simulink model "sm_wheel_loader_driveline"  (R2025a)
settings: Solver=VariableStepAuto  StartTime=0.0  StopTime=20  RelTol=1e-3  AbsTol=1e-3  EnableMultiTasking=on
undefined symbols (not defined in the file or in its folder): Wheel_Loader, X, Y, Z
libraries: sm_lib x12, sm_wheel_loader_lib x6, nesl_utility x3, fl_lib x3
Description:
  | Copyright 2023-2025 The MathWorks, Inc.
settings Model: Creator=smiller  LastModifiedBy=smiller
settings SolverCC: AutoScaleAbsTol=off  AlgebraicLoopSolver=TrustRegion  MaxZcPerStep=1.0
settings DataIOCC: LimitDataPoints=on  MaxDataPoints=10000  ReturnWorkspaceOutputs=off  SignalLoggingName=logsout_sm_wheel_loader_driveline
settings OptimizationCC: ReuseModelBlockBuffer=off  LifeSpan=inf
settings DebuggingCC: UnconnectedInputMsg=warning  UnconnectedOutputMsg=warning  UnconnectedLineMsg=warning  AllowSymbolicDim=off  SubsystemReferenceDiagnosticForUnitTest=warning  SFUnexpectedBacktrackingDiag=warning  SFNoUnconditionalDefaultTransitionDiag=warning  SFExecutionAtInitializationDiag=none  ArithmeticOperatorsInVariantConditions=warning
settings ModelReferenceCC: EnableRefExpFcnMdlSchedulingChecks=on
settings SFSimCC: SimUseLocalCustomCode=off  CustomCodeUndefinedFunction=UseInterfaceOnly
settings RTWCC: RTWUseLocalCustomCode=off  GPUComputeCapability=3.5  DLArmComputeVersion=19.05
settings CodeAppCC: StateflowObjectComments=on
settings GRTTargetCC: TargetLangStandard=C89/C90 (ANSI)
settings ConfigComp: CovMetricSettings=dw  CovSaveCumulativeToWorkspaceVar=on  CovSaveSingleToWorkspaceVar=on  CovExternalEMLEnable=off  CovSFcnEnable=off
settings SimscapeCC: SimscapeLogType=all  SimscapeLogSimulationStatistics=on  SimscapeLogName=simlog_sm_wheel_loader_driveline  SimscapeLogDataHistory=10000.0
settings DiagnosticsConfigSet: SimMechanicsUnconnectedFramePorts=none
settings ExplorerConfigSet: InternalSimMechanicsExplorerSettings="<ExplorerConfiguration><canonicalview>default</canonicalview><AnimationSetting><BasePlaybackSpeed>1.0</BasePlaybackSpeed><PlaybackSpeedFactor>1.0</PlaybackSpeedFactor></AnimationSetting><TilePanel><TileInfo><Tiles Columns=\"1\" Count=\"1\" Rows=\"1\"><Column Weight=\"1\"/><Row Weight=\"1\"/><Tile Height=\"1\" Width=\"1\" X=\"0\" Y=\"0\"/></Tiles></TileInfo><SceneInfo><SceneViewer><BGColor><R>1</R><G>1</G><B>1</B></BGColor><Camera><DoPerspective>off</DoPerspective><Position><X>-0.927464937859153515</X><Y>-0.882013825634648696</Y><Z>0.258089805407605677</Z></Position><Center><X>-0.254615293064785364</X><Y>-0.20835009329744858</Y><Z>-0.047606990836146286</Z></Center><Up><X>0.634087832148672037</X><Y>-0.738030275124983537</Y><Z>-0.230746471522185359</Z></Up><ViewLimDist>1</ViewLimDist><YLim>0.133380146481821338</YLim><XLim>0.282253946342844175</XLim></Camera></SceneViewer></SceneInfo></TilePanel><MechEditorPanel><Cameras/><GfxPanelCameraMap/><VideoCreator><PlaybackSpeedRatio>1.0</PlaybackSpeedRatio><FrameRate>30</FrameRate><VideoFormat>Motion JPEG AVI</VideoFormat><FrameSize>auto</FrameSize></VideoCreator></MechEditorPanel></ExplorerConfiguration>"

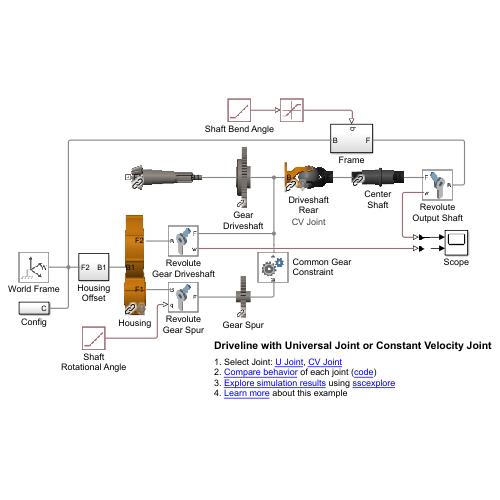
[thumbnail: Simulink's stored preview of the top-level diagram]
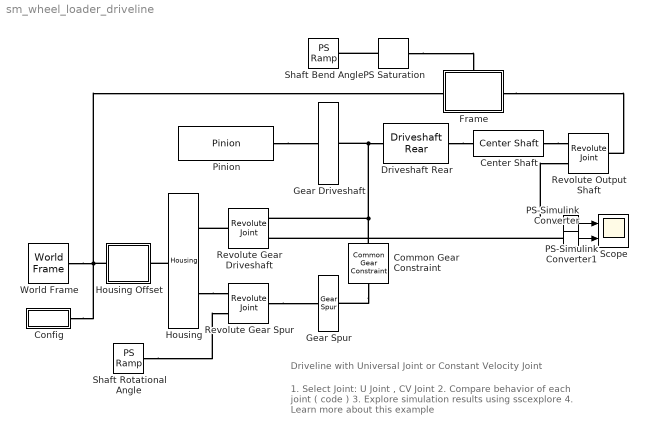
== system sm_wheel_loader_driveline ==
  note: Driveline with Universal Joint or Constant Velocity Joint
  note: 1. Select Joint: U Joint , CV Joint
      | 2. Compare behavior of each joint ( code )
      | 3. Explore simulation results using sscexplore
      | 4. Learn more about this example
  Center Shaft : sm_wheel_loader_lib/Wheel Loader Vehicle/Driveline/Driveline/Driveline 3D/Center Shaft  SystemSampleTime=-1  VariantActivationTime=update diagram  EmptyChoice=off  PassThrough=off  PassThroughVariantControl=(default)  EmptyChoiceVariantControl=(default)  AllowFlexibleInterface=on  Latency=0  AutoFrameSizeCalculation=off
  Common Gear Constraint : sm_lib/Gears and Couplings/Gears/Common Gear Constraint  GearType=External  SpecificationType=CenterDistanceRatio  CenterDistance=0.159173333333337  CenterDistanceUnits=m  GearRatio=60/34  BaseGearRadius=10.0  BaseGearRadiusUnits=cm  FollGearRadius=10.0  FollGearRadiusUnits=cm
  Config : Subsystem
  Driveshaft Rear : sm_wheel_loader_lib/Wheel Loader Vehicle/Driveline/Driveline/Driveline 3D/Driveshaft Rear  popup_driveJointR=CV Joint
      settings: AttributesFormatString=%<popup_driveJointR>
  Frame : Subsystem
      settings: PortSchema="{\"entries\":[{\"content\":{\"sides\":[{\"content\":{\"connectorIds\":[\"LConn1\"]},\"type\":\"ConnectorPlacement.EquallySpacedRectSide\",\"uuid\":\"e6cbbeaa-eea4-475d-99a8-9813de6a09fd\"},{\"content\":{\"connectorIds\":[\"RConn1\"],\"side\":\"RIGHT\"},\"type\":\"ConnectorPlacement.EquallySpacedRectSide\",\"uuid\":\"b42ffd92-551a-432a-a88e-4fe80a794cd4\"},{\"content\":{\"connectorIds\":[\"LConn2\"],\"side\":\"TOP\"},\"type\":\"ConnectorPlacement.EquallySpacedRectSide\",\"uuid\":\"5e4255e5-ca05-41fd-94c5-358a7ae7d752\"}]},\"type\":\"ConnectorPlacement.EquallySpacedConnector\",\"uuid\":\"ee1dc33c-92b2-4d9a-b7e0-7adfd33d81e9\"}],\"packageUris\":[\"http://schema.mathworks.com/mf0/Connector/R2020b\"],\"version\":\"1.0\"}"
  Gear Driveshaft : sm_wheel_loader_lib/Wheel Loader Vehicle/Driveline/Driveline/Driveline 3D/Gear Driveshaft  Tag=431AF5D6-54DA-7142-9431-C4596B630D74  SystemSampleTime=-1  VariantActivationTime=update diagram  EmptyChoice=off  PassThrough=off  PassThroughVariantControl=(default)  EmptyChoiceVariantControl=(default)  AllowFlexibleInterface=on  Latency=0  AutoFrameSizeCalculation=off
  Gear Spur : sm_wheel_loader_lib/Wheel Loader Vehicle/Driveline/Driveline/Driveline 3D/Gear Spur  Tag=6EB64544-2A1C-0847-BADC-74C9179BE488  SystemSampleTime=-1  VariantActivationTime=update diagram  EmptyChoice=off  PassThrough=off  PassThroughVariantControl=(default)  EmptyChoiceVariantControl=(default)  AllowFlexibleInterface=on  Latency=0  AutoFrameSizeCalculation=off
  Housing : sm_wheel_loader_lib/Wheel Loader Vehicle/Driveline/Driveline/Driveline 3D/Housing  Tag=FD1DF3FF-DA5A-0743-8F9C-61712535B657  finalDr_casing_opc=0.1
  Housing Offset : Subsystem
  PS Saturation : fl_lib/Physical Signals/Nonlinear Operators/PS Saturation  upper_limit=pi/4 rad  lower_limit=-pi/4 rad  ZeroCross=true
  PS-Simulink Converter : nesl_utility/PS-Simulink Converter  PhysicalDomain=network_engine_domain  SubClassName=ps_output  LeftPortType=input  RightPortType=output  PseudoPeriodic=off  Frequencies=[]  VectorFormat=inherit  Unit=inherit  AffineConversion=off
  PS-Simulink Converter1 : nesl_utility/PS-Simulink Converter  PhysicalDomain=network_engine_domain  SubClassName=ps_output  LeftPortType=input  RightPortType=output  PseudoPeriodic=off  Frequencies=[]  VectorFormat=inherit  Unit=inherit  AffineConversion=off
  Pinion : sm_wheel_loader_lib/Wheel Loader Vehicle/Driveline/Driveline/Driveline 3D/Pinion  Tag=8E104B94-12D7-814C-ADF4-87AC864C83F8  SystemSampleTime=-1  VariantActivationTime=update diagram  EmptyChoice=off  PassThrough=off  PassThroughVariantControl=(default)  EmptyChoiceVariantControl=(default)  AllowFlexibleInterface=on  Latency=0  AutoFrameSizeCalculation=off
  Revolute Gear Driveshaft : sm_lib/Joints/Revolute Joint  JointMode=Normal  CompositeWrenchDir=FollowerOnBase  CompositeWrenchFrame=BaseFrame  SenseConstraintForce=off  SenseConstraintTorque=off  SenseTotalForce=off  SenseTotalTorque=off  PositionTargetSpecify=off  PositionTargetPriority=High  PositionTargetValue=0  PositionTargetValueUnits=deg  VelocityTargetSpecify=off  VelocityTargetPriority=High  VelocityTargetValue=0  VelocityTargetValueUnits=deg/s  EquilibriumPosition=0  EquilibriumPositionUnits=deg  SpringStiffness=0  SpringStiffnessUnits=N*m/deg  DampingCoefficient=0  DampingCoefficientUnits=N*m/(deg/s)  LowerLimitSpecify=off  LowerLimitBound=-90  LowerLimitBoundUnits=deg  LowerLimitStiffness=1e4  LowerLimitStiffnessUnits=N*m/deg  LowerLimitDamping=10  LowerLimitDampingUnits=N*m/(deg/s)  LowerLimitTransitionRegionWidth=0.1  LowerLimitTransitionRegionWidthUnits=deg  UpperLimitSpecify=off  UpperLimitBound=90  UpperLimitBoundUnits=deg  UpperLimitStiffness=1e4  UpperLimitStiffnessUnits=N*m/deg  UpperLimitDamping=10  UpperLimitDampingUnits=N*m/(deg/s)  UpperLimitTransitionRegionWidth=0.1  UpperLimitTransitionRegionWidthUnits=deg  TorqueActuationMode=NoTorque  MotionActuationMode=ComputedMotion  SensePosition=off  SenseVelocity=on  SenseAcceleration=off  SenseTorqueForce=off  SenseLowerLimitTorqueForce=off  SenseUpperLimitTorqueForce=off
  Revolute Gear Spur : sm_lib/Joints/Revolute Joint  JointMode=Normal  CompositeWrenchDir=FollowerOnBase  CompositeWrenchFrame=BaseFrame  SenseConstraintForce=off  SenseConstraintTorque=off  SenseTotalForce=off  SenseTotalTorque=off  PositionTargetSpecify=off  PositionTargetPriority=High  PositionTargetValue=0  PositionTargetValueUnits=deg  VelocityTargetSpecify=off  VelocityTargetPriority=High  VelocityTargetValue=0  VelocityTargetValueUnits=deg/s  EquilibriumPosition=0  EquilibriumPositionUnits=deg  SpringStiffness=0  SpringStiffnessUnits=N*m/deg  DampingCoefficient=0  DampingCoefficientUnits=N*m/(deg/s)  LowerLimitSpecify=off  LowerLimitBound=-90  LowerLimitBoundUnits=deg  LowerLimitStiffness=1e4  LowerLimitStiffnessUnits=N*m/deg  LowerLimitDamping=10  LowerLimitDampingUnits=N*m/(deg/s)  LowerLimitTransitionRegionWidth=0.1  LowerLimitTransitionRegionWidthUnits=deg  UpperLimitSpecify=off  UpperLimitBound=90  UpperLimitBoundUnits=deg  UpperLimitStiffness=1e4  UpperLimitStiffnessUnits=N*m/deg  UpperLimitDamping=10  UpperLimitDampingUnits=N*m/(deg/s)  UpperLimitTransitionRegionWidth=0.1  UpperLimitTransitionRegionWidthUnits=deg  TorqueActuationMode=ComputedTorque  MotionActuationMode=InputMotion  SensePosition=off  SenseVelocity=off  SenseAcceleration=off  SenseTorqueForce=off  SenseLowerLimitTorqueForce=off  SenseUpperLimitTorqueForce=off
  Revolute Output Shaft : sm_lib/Joints/Revolute Joint  JointMode=Normal  CompositeWrenchDir=FollowerOnBase  CompositeWrenchFrame=BaseFrame  SenseConstraintForce=off  SenseConstraintTorque=off  SenseTotalForce=off  SenseTotalTorque=off  PositionTargetSpecify=off  PositionTargetPriority=High  PositionTargetValue=0  PositionTargetValueUnits=deg  VelocityTargetSpecify=off  VelocityTargetPriority=High  VelocityTargetValue=0  VelocityTargetValueUnits=deg/s  EquilibriumPosition=0  EquilibriumPositionUnits=deg  SpringStiffness=0  SpringStiffnessUnits=N*m/deg  DampingCoefficient=0  DampingCoefficientUnits=N*m/(deg/s)  LowerLimitSpecify=off  LowerLimitBound=-90  LowerLimitBoundUnits=deg  LowerLimitStiffness=1e4  LowerLimitStiffnessUnits=N*m/deg  LowerLimitDamping=10  LowerLimitDampingUnits=N*m/(deg/s)  LowerLimitTransitionRegionWidth=0.1  LowerLimitTransitionRegionWidthUnits=deg  UpperLimitSpecify=off  UpperLimitBound=90  UpperLimitBoundUnits=deg  UpperLimitStiffness=1e4  UpperLimitStiffnessUnits=N*m/deg  UpperLimitDamping=10  UpperLimitDampingUnits=N*m/(deg/s)  UpperLimitTransitionRegionWidth=0.1  UpperLimitTransitionRegionWidthUnits=deg  TorqueActuationMode=NoTorque  MotionActuationMode=ComputedMotion  SensePosition=off  SenseVelocity=on  SenseAcceleration=off  SenseTorqueForce=off  SenseLowerLimitTorqueForce=off  SenseUpperLimitTorqueForce=off
  Scope : Scope  NumInputPorts=2
      settings: ActiveDisplayYMinimum=-0.11127  ActiveDisplayYMaximum=1.0014
  Shaft Rotational Angle : fl_lib/Physical Signals/Sources/PS Ramp  slope=-15 rpm  start_time=0 s  initial_output=0  ZeroCross=true
  Shaft Bend Angle : fl_lib/Physical Signals/Sources/PS Ramp  slope=-pi/8 1/s  start_time=5 s  initial_output=0  ZeroCross=true
  World Frame : sm_lib/Frames and Transforms/World Frame
  wires:
  PS-Simulink Converter/1 -> Scope/2
  PS-Simulink Converter1/1 -> Scope/1
  connections:
  Housing/LConn1 -- Housing Offset/LConn1
  Common Gear Constraint/RConn1 -- Driveshaft Rear/LConn1 -- Gear Driveshaft/LConn1 -- Revolute Gear Driveshaft/RConn1
  Revolute Gear Spur/RConn1 -- Gear Spur/LConn1
  Common Gear Constraint/LConn1 -- Gear Spur/RConn1
  Driveshaft Rear/RConn1 -- Center Shaft/LConn1
  Housing/RConn2 -- Revolute Gear Spur/LConn1
  Revolute Gear Driveshaft/LConn1 -- Housing/RConn1
  Center Shaft/RConn1 -- Revolute Output Shaft/RConn1
  Shaft Rotational Angle/RConn1 -- Revolute Gear Spur/LConn2
  PS Saturation/LConn1 -- Shaft Bend Angle/RConn1
  PS-Simulink Converter/LConn1 -- Revolute Gear Driveshaft/RConn2
  PS-Simulink Converter1/LConn1 -- Revolute Output Shaft/RConn2
  Housing Offset/RConn1 -- World Frame/RConn1 -- Frame/LConn1 -- Config/RConn1
  Frame/RConn1 -- Revolute Output Shaft/LConn1
  PS Saturation/RConn1 -- Frame/LConn2
  Pinion/RConn1 -- Gear Driveshaft/RConn1

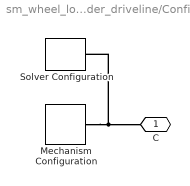
== system sm_wheel_loader_driveline/Config ==
  Mechanism Configuration : sm_lib/Utilities/Mechanism Configuration  UniformGravity=Constant  GravityVector=[0 0 -9.80665]  GravityVectorUnits=m/s^2  LinearizationDelta=0.001  JointModeTransitionNonlinearIterations=2
  Solver Configuration : nesl_utility/Solver Configuration  PhysicalDomain=network_engine_domain  SubClassName=solver  LeftPortType=input  RightPortType=generic  Tones=[]  Harmonics=[]  SimulateNoise=off  Profile=off  UseLocalSampling=off  EnableSwitchedLinearOptims=on  FrequencyDomain=off  UseCCode=off  RelTol=0.001  AbsTol=1e-06  MinStep=1e-09  ToWorkspace=off  RevertToSquareIcSolve=off  NumHomotopyIterations=100  PhasorMode=off  PhasorModeNumHarmonics=1  ConsistencySolver=NEWTON_XTOL_AFTER_FTOL  IndexReductionMethod=DerivativeReplacement  DoDC=off  ResidualTolerance=1e-09  ConsistencyTolSource=GLOBAL  ConsistencyAbsTol=0.001  ConsistencyRelTol=0.001  ConsistencyTolFactor=0.001  UseLocalSolver=off  LocalSolverChoice=NE_BACKWARD_EULER_ADVANCER  ResolveIndetEquations=on  FunctionEvalNumThread=1  LocalSolverSampleTime=0.001  DoFixedCost=off  MaxNonlinIter=3  MaxModeIter=2  ComputeImpulses=off  ImpulseIterations=2  LinearAlgebra=Sparse  LinearAlgebraNumThread=0  EquationFormulation=NE_TIME_EF  DelaysMemoryBudget=1024  AutomaticFiltering=on  FilteringTimeConstant=0.001  PartitionStorageMethod=AS_NEEDED  PartitionMemoryBudget=1024  PartitionMethod=FAST  MultibodyUseLocalSolver=off  MultibodyLocalSolverChoice=ODE1  MultibodyLocalSolverSampleTime=0.001
  C : PMIOPort  Side=Right
  connections:
  Mechanism Configuration/RConn1 -- Solver Configuration/RConn1 -- C/RConn1

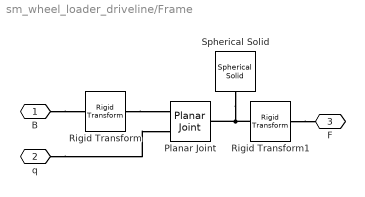
== system sm_wheel_loader_driveline/Frame ==
  Planar Joint : sm_lib/Joints/Planar Joint  JointMode=Normal  CompositeWrenchDir=FollowerOnBase  CompositeWrenchFrame=BaseFrame  SenseConstraintForce=off  SenseConstraintTorque=off  SenseTotalForce=off  SenseTotalTorque=off  PxPositionTargetSpecify=off  PxPositionTargetPriority=High  PxPositionTargetValue=0  PxPositionTargetValueUnits=m  PxVelocityTargetSpecify=off  PxVelocityTargetPriority=High  PxVelocityTargetValue=0  PxVelocityTargetValueUnits=m/s  PxEquilibriumPosition=0  PxEquilibriumPositionUnits=m  PxSpringStiffness=0  PxSpringStiffnessUnits=N/m  PxDampingCoefficient=0  PxDampingCoefficientUnits=N/(m/s)  PxLowerLimitSpecify=off  PxLowerLimitBound=-1  PxLowerLimitBoundUnits=m  PxLowerLimitStiffness=1e6  PxLowerLimitStiffnessUnits=N/m  PxLowerLimitDamping=1e3  PxLowerLimitDampingUnits=N/(m/s)  PxLowerLimitTransitionRegionWidth=1e-4  PxLowerLimitTransitionRegionWidthUnits=m  PxUpperLimitSpecify=off  PxUpperLimitBound=1  PxUpperLimitBoundUnits=m  PxUpperLimitStiffness=1e6  PxUpperLimitStiffnessUnits=N/m  PxUpperLimitDamping=1e3  PxUpperLimitDampingUnits=N/(m/s)  PxUpperLimitTransitionRegionWidth=1e-4  PxUpperLimitTransitionRegionWidthUnits=m  PxTorqueActuationMode=NoTorque  PxMotionActuationMode=ComputedMotion  PxSensePosition=off  PxSenseVelocity=off  PxSenseAcceleration=off  PxSenseTorqueForce=off  PxSenseLowerLimitTorqueForce=off  PxSenseUpperLimitTorqueForce=off  PyPositionTargetSpecify=off  PyPositionTargetPriority=High  PyPositionTargetValue=0  PyPositionTargetValueUnits=m  PyVelocityTargetSpecify=off  PyVelocityTargetPriority=High  PyVelocityTargetValue=0  PyVelocityTargetValueUnits=m/s  PyEquilibriumPosition=0  PyEquilibriumPositionUnits=m  PySpringStiffness=0  PySpringStiffnessUnits=N/m  PyDampingCoefficient=0  PyDampingCoefficientUnits=N/(m/s)  PyLowerLimitSpecify=off  PyLowerLimitBound=-1  PyLowerLimitBoundUnits=m  PyLowerLimitStiffness=1e6  PyLowerLimitStiffnessUnits=N/m  PyLowerLimitDamping=1e3  PyLowerLimitDampingUnits=N/(m/s)  PyLowerLimitTransitionRegionWidth=1e-4  PyLowerLimitTransitionRegionWidthUnits=m  PyUpperLimitSpecify=off  PyUpperLimitBound=1  PyUpperLimitBoundUnits=m  PyUpperLimitStiffness=1e6  PyUpperLimitStiffnessUnits=N/m  PyUpperLimitDamping=1e3  PyUpperLimitDampingUnits=N/(m/s)  PyUpperLimitTransitionRegionWidth=1e-4  PyUpperLimitTransitionRegionWidthUnits=m  PyTorqueActuationMode=NoTorque  PyMotionActuationMode=ComputedMotion  PySensePosition=off  PySenseVelocity=off  PySenseAcceleration=off  PySenseTorqueForce=off  PySenseLowerLimitTorqueForce=off  PySenseUpperLimitTorqueForce=off  RzPositionTargetSpecify=off  RzPositionTargetPriority=High  RzPositionTargetValue=0  RzPositionTargetValueUnits=deg  RzVelocityTargetSpecify=off  RzVelocityTargetPriority=High  RzVelocityTargetValue=0  RzVelocityTargetValueUnits=deg/s  RzEquilibriumPosition=0  RzEquilibriumPositionUnits=deg  RzSpringStiffness=0  RzSpringStiffnessUnits=N*m/deg  RzDampingCoefficient=0  RzDampingCoefficientUnits=N*m/(deg/s)  RzLowerLimitSpecify=off  RzLowerLimitBound=-90  RzLowerLimitBoundUnits=deg  RzLowerLimitStiffness=1e4  RzLowerLimitStiffnessUnits=N*m/deg  RzLowerLimitDamping=10  RzLowerLimitDampingUnits=N*m/(deg/s)  RzLowerLimitTransitionRegionWidth=0.1  RzLowerLimitTransitionRegionWidthUnits=deg  RzUpperLimitSpecify=off  RzUpperLimitBound=90  RzUpperLimitBoundUnits=deg  RzUpperLimitStiffness=1e4  RzUpperLimitStiffnessUnits=N*m/deg  RzUpperLimitDamping=10  RzUpperLimitDampingUnits=N*m/(deg/s)  RzUpperLimitTransitionRegionWidth=0.1  RzUpperLimitTransitionRegionWidthUnits=deg  RzTorqueActuationMode=ComputedTorque  RzMotionActuationMode=InputMotion  RzSensePosition=off  RzSenseVelocity=off  RzSenseAcceleration=off  RzSenseTorqueForce=off  RzSenseLowerLimitTorqueForce=off  RzSenseUpperLimitTorqueForce=off
  Rigid Transform : sm_lib/Frames and Transforms/Rigid Transform  RotationMethod=StandardAxis  FollAlignAxisA=+X  BaseAlignAxisA=+Y  FollAlignAxisB=+Y  BaseAlignAxisB=+Z  RotationStandardAxis=+X  RotationAngle=90  RotationAngleUnits=deg  RotationArbitraryAxis=[0 0 1]  RotationSequenceAxes=FollowerAxes  RotationSequence=XYX  RotationSequenceAngles=[0 0 0]  RotationSequenceAnglesUnits=deg  RotationMatrix=[1 0 0; 0 1 0; 0 0 1]  Quaternion=[1 0 0 0]  TranslationMethod=None  TranslationCartesianOffset=[0 0 0]  TranslationCartesianOffsetUnits=m  TranslationStandardAxis=+Z  TranslationStandardOffset=0  TranslationStandardOffsetUnits=m  TranslationROffset=0  TranslationROffsetUnits=m  TranslationThetaOffset=0  TranslationThetaOffsetUnits=deg  TranslationZOffset=0  TranslationZOffsetUnits=m
  Rigid Transform1 : sm_lib/Frames and Transforms/Rigid Transform  RotationMethod=StandardAxis  FollAlignAxisA=+X  BaseAlignAxisA=+Y  FollAlignAxisB=+Y  BaseAlignAxisB=+Z  RotationStandardAxis=+X  RotationAngle=90  RotationAngleUnits=deg  RotationArbitraryAxis=[0 0 1]  RotationSequenceAxes=FollowerAxes  RotationSequence=XYX  RotationSequenceAngles=[0 0 0]  RotationSequenceAnglesUnits=deg  RotationMatrix=[1 0 0; 0 1 0; 0 0 1]  Quaternion=[1 0 0 0]  TranslationMethod=None  TranslationCartesianOffset=[0 0 0]  TranslationCartesianOffsetUnits=m  TranslationStandardAxis=+Z  TranslationStandardOffset=0  TranslationStandardOffsetUnits=m  TranslationROffset=0  TranslationROffsetUnits=m  TranslationThetaOffset=0  TranslationThetaOffsetUnits=deg  TranslationZOffset=0  TranslationZOffsetUnits=m
  Spherical Solid : sm_lib/Body Elements/Spherical Solid  SphereRadius=0.01  SphereRadiusUnits=m  ExportEntireGeometry=off  InertiaType=CalculateFromGeometry  BasedOnType=Density  Density=1000  DensityUnits=kg/m^3  Mass=1  MassUnits=kg  CenterOfMass=[0 0 0]  CenterOfMassUnits=m  MomentsOfInertia=[1 1 1]  MomentsOfInertiaUnits=kg*m^2  ProductsOfInertia=[0 0 0]  ProductsOfInertiaUnits=kg*m^2  GraphicType=FromGeometry  MarkerShape=Sphere  MarkerSize=10  GraphicVisPropType=SimpleVisualProperties  GraphicDiffuseColor=[0.5 0.5 0.5]  GraphicOpacity=1.0  GraphicSpecularColor=[0.5 0.5 0.5 1.0]  GraphicAmbientColor=[0.15 0.15 0.15 1.0]  GraphicEmissiveColor=[0.0 0.0 0.0 1.0]  GraphicShininess=75  DoExposeReferenceFrame=on  SerializedFrames=<Frames/>
  B : PMIOPort  Side=Left
  q : PMIOPort  Port=2  Side=Left
  F : PMIOPort  Port=3  Side=Right
  connections:
  Rigid Transform/RConn1 -- Planar Joint/LConn1
  Rigid Transform1/RConn1 -- Spherical Solid/RConn1 -- Planar Joint/RConn1
  q/RConn1 -- Planar Joint/LConn2
  Rigid Transform1/LConn1 -- F/RConn1
  B/RConn1 -- Rigid Transform/LConn1

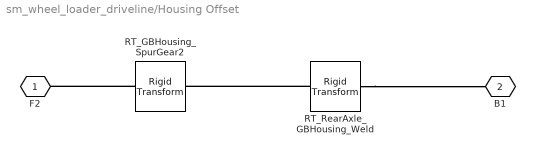
== system sm_wheel_loader_driveline/Housing Offset ==
  RT_GBHousing_SpurGear2 : sm_lib/Frames and Transforms/Rigid Transform  RotationMethod=RotationMatrix  FollAlignAxisA=+X  BaseAlignAxisA=+Y  FollAlignAxisB=+Y  BaseAlignAxisB=+Z  RotationStandardAxis=+Z  RotationAngle=0.0  RotationAngleUnits=deg  RotationArbitraryAxis=[0 0 1]  RotationSequenceAxes=FollowerAxes  RotationSequence=XYX  RotationSequenceAngles=[0 0 0]  RotationSequenceAnglesUnits=deg  RotationMatrix=Wheel_Loader.coordSys(55).transform.rotation  Quaternion=[1 0 0 0]  TranslationMethod=Cartesian  TranslationCartesianOffset=Wheel_Loader.coordSys(55).transform.translation  TranslationCartesianOffsetUnits=m  TranslationStandardAxis=+Z  TranslationStandardOffset=0  TranslationStandardOffsetUnits=m  TranslationROffset=0  TranslationROffsetUnits=m  TranslationThetaOffset=0  TranslationThetaOffsetUnits=deg  TranslationZOffset=0  TranslationZOffsetUnits=m
  RT_RearAxle_GBHousing_Weld : sm_lib/Frames and Transforms/Rigid Transform  RotationMethod=RotationMatrix  FollAlignAxisA=+X  BaseAlignAxisA=+Y  FollAlignAxisB=+Y  BaseAlignAxisB=+Z  RotationStandardAxis=+Z  RotationAngle=0.0  RotationAngleUnits=deg  RotationArbitraryAxis=[0 0 1]  RotationSequenceAxes=FollowerAxes  RotationSequence=XYX  RotationSequenceAngles=[0 0 0]  RotationSequenceAnglesUnits=deg  RotationMatrix=Wheel_Loader.coordSys(56).transform.rotation  Quaternion=[1 0 0 0]  TranslationMethod=Cartesian  TranslationCartesianOffset=Wheel_Loader.coordSys(56).transform.translation  TranslationCartesianOffsetUnits=m  TranslationStandardAxis=+Z  TranslationStandardOffset=0  TranslationStandardOffsetUnits=m  TranslationROffset=0  TranslationROffsetUnits=m  TranslationThetaOffset=0  TranslationThetaOffsetUnits=deg  TranslationZOffset=0  TranslationZOffsetUnits=m
  F2 : PMIOPort  Side=Right
  B1 : PMIOPort  Port=2  Side=Left
  connections:
  RT_GBHousing_SpurGear2/RConn1 -- F2/RConn1
  RT_RearAxle_GBHousing_Weld/LConn1 -- RT_GBHousing_SpurGear2/LConn1
  RT_RearAxle_GBHousing_Weld/RConn1 -- B1/RConn1
